simulink model "Swerve_Drive_Example_Model"  (R2023b)
settings: Solver=daessc  StartTime=0.0  StopTime=10  FixedStep=t_sample  RelTol=1e-3
undefined symbols (not defined in the file or in its folder): t_sample
libraries: SignalEditorBlockLib x1, Simulation_lib x1
settings Model: SimulationMode=accelerator  Creator=ander  LastModifiedBy=ander

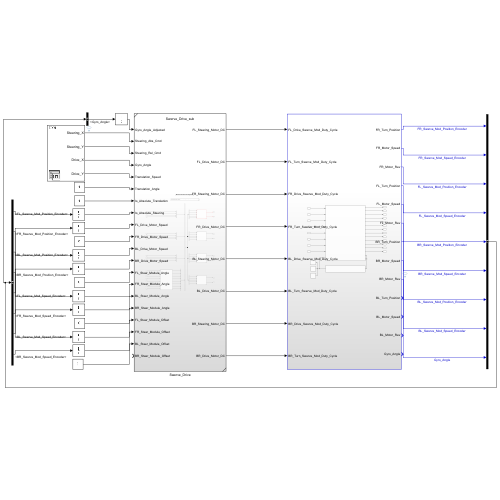
[thumbnail: Simulink's stored preview of the top-level diagram]
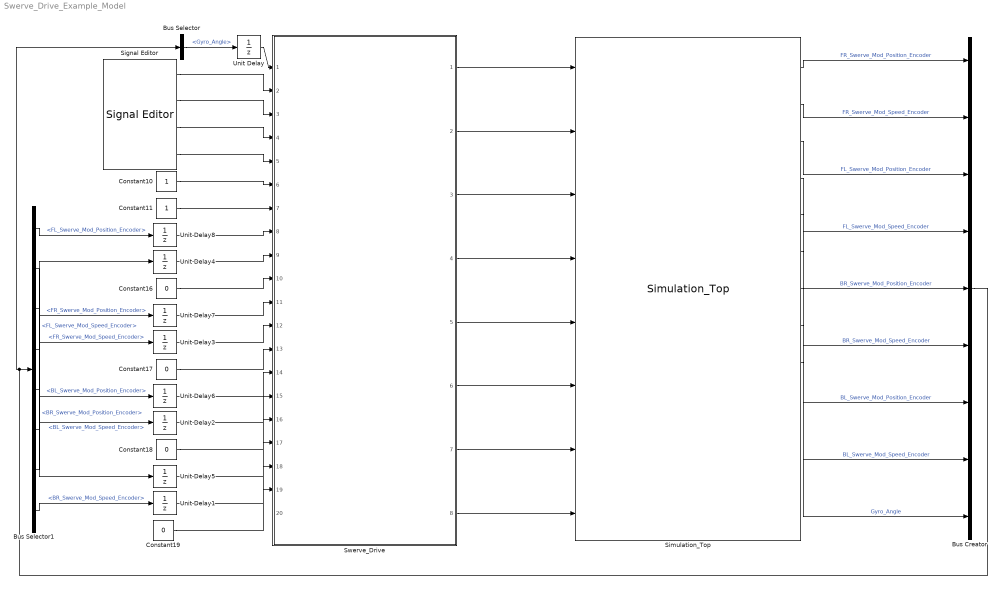
== system Swerve_Drive_Example_Model ==
  Bus Creator : BusCreator  Inputs=9
  Bus Selector : BusSelector  OutputSignals=Gyro_Angle
  Bus Selector1 : BusSelector  OutputSignals=FL_Swerve_Mod_Position_Encoder,FR_Swerve_Mod_Position_Encoder,BL_Swerve_Mod_Position_Encoder,BR_Swerve_Mod_Position_Encoder,FL_Swerve_Mod_Speed_Encoder,FR_Swerve_Mod_Speed_Encoder,BL_Swerve_Mod_Speed_Encoder,BR_Swerve_Mod_Speed_Encoder
  Constant10 : Constant  OutDataTypeStr=boolean
  Constant11 : Constant  OutDataTypeStr=boolean
  Constant{16..19} (4 alike) : Constant  Value=0
  Signal Editor : SignalEditorBlockLib/Signal Editor  FileName=Joystick_input_test_data.mat  ActiveScenario=DXN  ActiveSignal=Drive_X  IsBus=off  OutputBusObjectStr=Bus: BusObject  SampleTime=t_sample  ZeroCross=off  OutputAfterFinalValue=Setting to zero  Unit=inherit  PreserveSignalName=on  ApplySigPropsToAllScenarios=on  ApplySigPropsToAllSignals=off
  Simulation_Top : Simulation_lib/Simulation_Top  SystemSampleTime=-1  VariantActivationTime=update diagram  AllowFlexibleInterface=on  Latency=0  AutoFrameSizeCalculation=off
  Swerve_Drive : Subsystem  ReferencedSubsystem=Swerve_Drive_sub
  Unit Delay{,1..8} (9 alike) : UnitDelay  SampleTime=-1  HasFrameUpgradeWarning=on
  wires:
  Constant11/1 -> Swerve_Drive/7
  Constant10/1 -> Swerve_Drive/6
  Constant17/1 -> Swerve_Drive/13
  Constant19/1 -> Swerve_Drive/19
  Constant16/1 -> Swerve_Drive/10
  Constant18/1 -> Swerve_Drive/16
  Unit Delay/1 -> Swerve_Drive/1
  Unit Delay1/1 -> Swerve_Drive/18
  Unit Delay2/1 -> Swerve_Drive/15
  Unit Delay3/1 -> Swerve_Drive/12
  Simulation_Top/9 -> Bus Creator/9  "Gyro_Angle"
  Simulation_Top/8 -> Bus Creator/8  "BL_Swerve_Mod_Speed_Encoder"
  Simulation_Top/7 -> Bus Creator/7  "BL_Swerve_Mod_Position_Encoder"
  Simulation_Top/6 -> Bus Creator/6  "BR_Swerve_Mod_Speed_Encoder"
  Simulation_Top/5 -> Bus Creator/5  "BR_Swerve_Mod_Position_Encoder"
  Simulation_Top/4 -> Bus Creator/4  "FL_Swerve_Mod_Speed_Encoder"
  Simulation_Top/3 -> Bus Creator/3  "FL_Swerve_Mod_Position_Encoder"
  Simulation_Top/2 -> Bus Creator/2  "FR_Swerve_Mod_Speed_Encoder"
  Simulation_Top/1 -> Bus Creator/1  "FR_Swerve_Mod_Position_Encoder"
  Swerve_Drive/1 -> Simulation_Top/1
  Swerve_Drive/2 -> Simulation_Top/2
  Swerve_Drive/3 -> Simulation_Top/3
  Swerve_Drive/4 -> Simulation_Top/4
  Swerve_Drive/5 -> Simulation_Top/5
  Swerve_Drive/6 -> Simulation_Top/6
  Swerve_Drive/7 -> Simulation_Top/7
  Swerve_Drive/8 -> Simulation_Top/8
  Bus Selector/1 -> Unit Delay/1  "<Gyro_Angle>"
  Bus Creator/1 -> Bus Selector/1, Bus Selector1/1
  Bus Selector1/1 -> Unit Delay8/1  "<FL_Swerve_Mod_Position_Encoder>"
  Bus Selector1/2 -> Unit Delay7/1  "<FR_Swerve_Mod_Position_Encoder>"
  Bus Selector1/3 -> Unit Delay6/1  "<BL_Swerve_Mod_Position_Encoder>"
  Bus Selector1/4 -> Unit Delay5/1  "<BR_Swerve_Mod_Position_Encoder>"
  Bus Selector1/5 -> Unit Delay4/1  "<FL_Swerve_Mod_Speed_Encoder>"
  Bus Selector1/6 -> Unit Delay3/1  "<FR_Swerve_Mod_Speed_Encoder>"
  Bus Selector1/7 -> Unit Delay2/1  "<BL_Swerve_Mod_Speed_Encoder>"
  Bus Selector1/8 -> Unit Delay1/1  "<BR_Swerve_Mod_Speed_Encoder>"
  Signal Editor/4 -> Swerve_Drive/5
  Signal Editor/3 -> Swerve_Drive/4
  Signal Editor/2 -> Swerve_Drive/3
  Signal Editor/1 -> Swerve_Drive/2
  Unit Delay8/1 -> Swerve_Drive/8
  Unit Delay7/1 -> Swerve_Drive/11
  Unit Delay6/1 -> Swerve_Drive/14
  Unit Delay5/1 -> Swerve_Drive/17
  Unit Delay4/1 -> Swerve_Drive/9
